simulink model "DCHR_A40_Safety_Controller"  (R2026a)
settings: Solver=FixedStepDiscrete  StopTime=603900  FixedStep=900
settings Model: Creator=Lysda  LastModifiedBy=Lysda

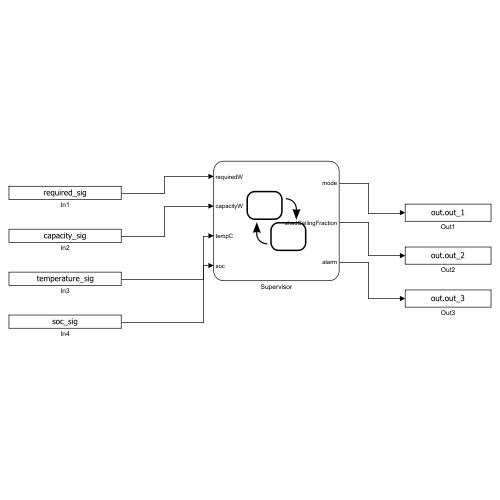
[thumbnail: Simulink's stored preview of the top-level diagram]
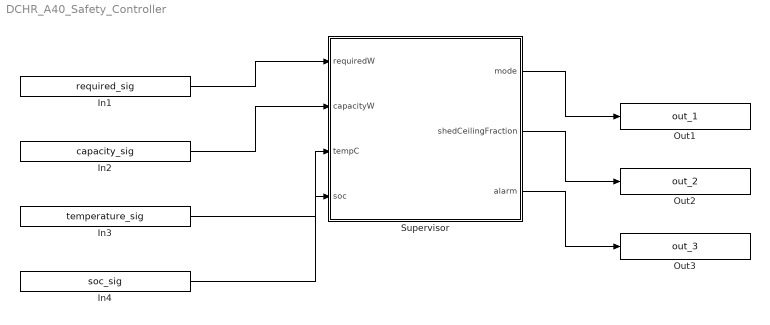
== system DCHR_A40_Safety_Controller ==
  In1 : FromWorkspace  VariableName=required_sig
  In2 : FromWorkspace  VariableName=capacity_sig
  In3 : FromWorkspace  VariableName=temperature_sig
  In4 : FromWorkspace  VariableName=soc_sig
  Out1 : ToWorkspace  VariableName=out_1  SampleTime=-1
  Out2 : ToWorkspace  VariableName=out_2  SampleTime=-1
  Out3 : ToWorkspace  VariableName=out_3  SampleTime=-1
  Supervisor : Stateflow chart  TreatAsAtomicUnit=on
  wires:
  In1/1 -> Supervisor/1(requiredW)
  In2/1 -> Supervisor/2(capacityW)
  In3/1 -> Supervisor/3(tempC)
  In4/1 -> Supervisor/4(soc)
  Supervisor/1(mode) -> Out1/1
  Supervisor/2(shedCeilingFraction) -> Out2/1
  Supervisor/3(alarm) -> Out3/1

== stateflow chart DCHR_A40_Safety_Controller/Supervisor ==
  state NORMAL
    entry: mode=0; shedCeilingFraction=0; alarm=0;
  state DEGRADED
    entry: mode=1; shedCeilingFraction=0.4; alarm=1;
  state TES_FULL
    entry: mode=3; shedCeilingFraction=0; alarm=1;
  state CRITICAL
    entry: mode=2; shedCeilingFraction=0.4; alarm=2;
  DEGRADED -> NORMAL [order 2] : [requiredW + 5000 <= capacityW && tempC < 39 && soc < 0.999]
  (default) -> NORMAL
  TES_FULL -> NORMAL [order 1] : [soc <= 0.98 && requiredW + 5000 <= capacityW && tempC < 39]
  DEGRADED -> TES_FULL [order 3] : [soc >= 0.999 && requiredW + 5000 <= capacityW && tempC < 39]
  TES_FULL -> DEGRADED [order 2] : [requiredW > capacityW + 1e-6 && tempC < 42 && capacityW > 0]
  NORMAL -> DEGRADED [order 1] : [requiredW > capacityW + 1e-6 && tempC < 42 && capacityW > 0]
  CRITICAL -> DEGRADED : [tempC < 39 && capacityW > 0]
  NORMAL -> CRITICAL [order 2] : [tempC >= 42 || capacityW <= 0]
  NORMAL -> TES_FULL [order 3] : [soc >= 0.999 && requiredW <= capacityW && tempC < 42 && capacityW > 0]
  DEGRADED -> CRITICAL [order 1] : [tempC >= 42 || capacityW <= 0]
  TES_FULL -> CRITICAL [order 3] : [tempC >= 42 || capacityW <= 0]
  data: requiredW input; capacityW input; tempC input; soc input; mode output; shedCeilingFraction output; alarm output
